simulink model "xz_packaging_automatic"  (R2025b)
settings: Solver=ode15s  StartTime=0.0  StopTime=13.05  MaxStep=0.001  RelTol=1e-6  AbsTol=1e-9
model workspace: external: MATLAB File xz_packaging_automatic_DataFile.m (data not in the file)
values from neighbouring files (symbols this model uses):
  payloadMass_kg = 0.25    [xz_packaging_automatic_DataFile.m]
undefined symbols (not defined in the file or in its folder): smiData, X, Y, Z
libraries: sm_lib x2549, nesl_utility x31
(part 37 of 38)

== system xz_packaging_automatic/Z_AXIS_ELGC_BS_45_200/RigidSubsystem/Z_GUIDE_FIXED_MOUNTS_RIGID/Z_GUIDE_FIXED_MOUNTS_1_RIGID/Z_FGUIDE_RIGHT_FOOT_WASH_1_LOW_RIGID ==
  ReferenceFrame : sm_lib/Frames and Transforms/Reference Frame
  Solid : sm_lib/Body Elements/File Solid  ExtGeomFileName=z_fguide_right_foot_wash_1_low_prt.step  UnitType=FromFile  ExtGeomFileUnits=m  StepReaderType=HEX  ExportConvexHullGeometry=off  InertiaType=Custom  BasedOnType=DensityFromFile  Density=1000  DensityUnits=kg/m^3  Mass=smiData.Solid(88).mass  MassUnits=kg  CenterOfMass=smiData.Solid(88).CoM  CenterOfMassUnits=mm  MomentsOfInertia=smiData.Solid(88).MoI  MomentsOfInertiaUnits=kg*mm^2  ProductsOfInertia=smiData.Solid(88).PoI  ProductsOfInertiaUnits=kg*mm^2  GraphicType=FromGeometry  MarkerShape=Sphere  MarkerSize=10  GraphicVisPropType=SimpleVisualProperties  GraphicDiffuseColor=smiData.Solid(88).color  GraphicOpacity=smiData.Solid(88).opacity  GraphicSpecularColor=[0.5 0.5 0.5 1.0]  GraphicAmbientColor=[0.15 0.15 0.15 1.0]  GraphicEmissiveColor=[0.0 0.0 0.0 1.0]  GraphicShininess=75  DoExposeReferenceFrame=on  SerializedFrames=<Frames/>
  F : PMIOPort  Side=Left
  connections:
  Solid/RConn1 -- ReferenceFrame/RConn1 -- F/RConn1

== system xz_packaging_automatic/Z_AXIS_ELGC_BS_45_200/RigidSubsystem/Z_GUIDE_FIXED_MOUNTS_RIGID/Z_GUIDE_FIXED_MOUNTS_1_RIGID/Z_FGUIDE_RIGHT_FOOT_WASH_1_TOP_RIGID ==
  ReferenceFrame : sm_lib/Frames and Transforms/Reference Frame
  Solid : sm_lib/Body Elements/File Solid  ExtGeomFileName=z_fguide_right_foot_wash_1_top_prt.step  UnitType=FromFile  ExtGeomFileUnits=m  StepReaderType=HEX  ExportConvexHullGeometry=off  InertiaType=Custom  BasedOnType=DensityFromFile  Density=1000  DensityUnits=kg/m^3  Mass=smiData.Solid(87).mass  MassUnits=kg  CenterOfMass=smiData.Solid(87).CoM  CenterOfMassUnits=mm  MomentsOfInertia=smiData.Solid(87).MoI  MomentsOfInertiaUnits=kg*mm^2  ProductsOfInertia=smiData.Solid(87).PoI  ProductsOfInertiaUnits=kg*mm^2  GraphicType=FromGeometry  MarkerShape=Sphere  MarkerSize=10  GraphicVisPropType=SimpleVisualProperties  GraphicDiffuseColor=smiData.Solid(87).color  GraphicOpacity=smiData.Solid(87).opacity  GraphicSpecularColor=[0.5 0.5 0.5 1.0]  GraphicAmbientColor=[0.15 0.15 0.15 1.0]  GraphicEmissiveColor=[0.0 0.0 0.0 1.0]  GraphicShininess=75  DoExposeReferenceFrame=on  SerializedFrames=<Frames/>
  F : PMIOPort  Side=Left
  connections:
  Solid/RConn1 -- ReferenceFrame/RConn1 -- F/RConn1

== system xz_packaging_automatic/Z_AXIS_ELGC_BS_45_200/RigidSubsystem/Z_GUIDE_FIXED_MOUNTS_RIGID/Z_GUIDE_FIXED_MOUNTS_1_RIGID/Z_FGUIDE_RIGHT_FOOT_WASH_2_LOW_RIGID ==
  ReferenceFrame : sm_lib/Frames and Transforms/Reference Frame
  Solid : sm_lib/Body Elements/File Solid  ExtGeomFileName=z_fguide_right_foot_wash_2_low_prt.step  UnitType=FromFile  ExtGeomFileUnits=m  StepReaderType=HEX  ExportConvexHullGeometry=off  InertiaType=Custom  BasedOnType=DensityFromFile  Density=1000  DensityUnits=kg/m^3  Mass=smiData.Solid(96).mass  MassUnits=kg  CenterOfMass=smiData.Solid(96).CoM  CenterOfMassUnits=mm  MomentsOfInertia=smiData.Solid(96).MoI  MomentsOfInertiaUnits=kg*mm^2  ProductsOfInertia=smiData.Solid(96).PoI  ProductsOfInertiaUnits=kg*mm^2  GraphicType=FromGeometry  MarkerShape=Sphere  MarkerSize=10  GraphicVisPropType=SimpleVisualProperties  GraphicDiffuseColor=smiData.Solid(96).color  GraphicOpacity=smiData.Solid(96).opacity  GraphicSpecularColor=[0.5 0.5 0.5 1.0]  GraphicAmbientColor=[0.15 0.15 0.15 1.0]  GraphicEmissiveColor=[0.0 0.0 0.0 1.0]  GraphicShininess=75  DoExposeReferenceFrame=on  SerializedFrames=<Frames/>
  F : PMIOPort  Side=Left
  connections:
  Solid/RConn1 -- ReferenceFrame/RConn1 -- F/RConn1

== system xz_packaging_automatic/Z_AXIS_ELGC_BS_45_200/RigidSubsystem/Z_GUIDE_FIXED_MOUNTS_RIGID/Z_GUIDE_FIXED_MOUNTS_1_RIGID/Z_FGUIDE_RIGHT_FOOT_WASH_2_TOP_RIGID ==
  ReferenceFrame : sm_lib/Frames and Transforms/Reference Frame
  Solid : sm_lib/Body Elements/File Solid  ExtGeomFileName=z_fguide_right_foot_wash_2_top_prt.step  UnitType=FromFile  ExtGeomFileUnits=m  StepReaderType=HEX  ExportConvexHullGeometry=off  InertiaType=Custom  BasedOnType=DensityFromFile  Density=1000  DensityUnits=kg/m^3  Mass=smiData.Solid(95).mass  MassUnits=kg  CenterOfMass=smiData.Solid(95).CoM  CenterOfMassUnits=mm  MomentsOfInertia=smiData.Solid(95).MoI  MomentsOfInertiaUnits=kg*mm^2  ProductsOfInertia=smiData.Solid(95).PoI  ProductsOfInertiaUnits=kg*mm^2  GraphicType=FromGeometry  MarkerShape=Sphere  MarkerSize=10  GraphicVisPropType=SimpleVisualProperties  GraphicDiffuseColor=smiData.Solid(95).color  GraphicOpacity=smiData.Solid(95).opacity  GraphicSpecularColor=[0.5 0.5 0.5 1.0]  GraphicAmbientColor=[0.15 0.15 0.15 1.0]  GraphicEmissiveColor=[0.0 0.0 0.0 1.0]  GraphicShininess=75  DoExposeReferenceFrame=on  SerializedFrames=<Frames/>
  F : PMIOPort  Side=Left
  connections:
  Solid/RConn1 -- ReferenceFrame/RConn1 -- F/RConn1

== system xz_packaging_automatic/Z_AXIS_ELGC_BS_45_200/RigidSubsystem/Z_GUIDE_FIXED_MOUNTS_RIGID/Z_GUIDE_FIXED_MOUNTS_1_RIGID/Z_FGUIDE_RIGHT_WALL_BOLT_1_M3X1_RIGID ==
  ReferenceFrame : sm_lib/Frames and Transforms/Reference Frame
  Solid : sm_lib/Body Elements/File Solid  ExtGeomFileName=z_fguide_right_wall_bolt_1_m3x1_prt.step  UnitType=FromFile  ExtGeomFileUnits=m  StepReaderType=HEX  ExportConvexHullGeometry=off  InertiaType=Custom  BasedOnType=DensityFromFile  Density=1000  DensityUnits=kg/m^3  Mass=smiData.Solid(90).mass  MassUnits=kg  CenterOfMass=smiData.Solid(90).CoM  CenterOfMassUnits=mm  MomentsOfInertia=smiData.Solid(90).MoI  MomentsOfInertiaUnits=kg*mm^2  ProductsOfInertia=smiData.Solid(90).PoI  ProductsOfInertiaUnits=kg*mm^2  GraphicType=FromGeometry  MarkerShape=Sphere  MarkerSize=10  GraphicVisPropType=SimpleVisualProperties  GraphicDiffuseColor=smiData.Solid(90).color  GraphicOpacity=smiData.Solid(90).opacity  GraphicSpecularColor=[0.5 0.5 0.5 1.0]  GraphicAmbientColor=[0.15 0.15 0.15 1.0]  GraphicEmissiveColor=[0.0 0.0 0.0 1.0]  GraphicShininess=75  DoExposeReferenceFrame=on  SerializedFrames=<Frames/>
  F : PMIOPort  Side=Left
  connections:
  Solid/RConn1 -- ReferenceFrame/RConn1 -- F/RConn1

== system xz_packaging_automatic/Z_AXIS_ELGC_BS_45_200/RigidSubsystem/Z_GUIDE_FIXED_MOUNTS_RIGID/Z_GUIDE_FIXED_MOUNTS_1_RIGID/Z_FGUIDE_RIGHT_WALL_BOLT_2_M3X1_RIGID ==
  ReferenceFrame : sm_lib/Frames and Transforms/Reference Frame
  Solid : sm_lib/Body Elements/File Solid  ExtGeomFileName=z_fguide_right_wall_bolt_2_m3x1_prt.step  UnitType=FromFile  ExtGeomFileUnits=m  StepReaderType=HEX  ExportConvexHullGeometry=off  InertiaType=Custom  BasedOnType=DensityFromFile  Density=1000  DensityUnits=kg/m^3  Mass=smiData.Solid(98).mass  MassUnits=kg  CenterOfMass=smiData.Solid(98).CoM  CenterOfMassUnits=mm  MomentsOfInertia=smiData.Solid(98).MoI  MomentsOfInertiaUnits=kg*mm^2  ProductsOfInertia=smiData.Solid(98).PoI  ProductsOfInertiaUnits=kg*mm^2  GraphicType=FromGeometry  MarkerShape=Sphere  MarkerSize=10  GraphicVisPropType=SimpleVisualProperties  GraphicDiffuseColor=smiData.Solid(98).color  GraphicOpacity=smiData.Solid(98).opacity  GraphicSpecularColor=[0.5 0.5 0.5 1.0]  GraphicAmbientColor=[0.15 0.15 0.15 1.0]  GraphicEmissiveColor=[0.0 0.0 0.0 1.0]  GraphicShininess=75  DoExposeReferenceFrame=on  SerializedFrames=<Frames/>
  F : PMIOPort  Side=Left
  connections:
  Solid/RConn1 -- ReferenceFrame/RConn1 -- F/RConn1

== system xz_packaging_automatic/Z_AXIS_ELGC_BS_45_200/RigidSubsystem/Z_GUIDE_FIXED_MOUNTS_RIGID/Z_GUIDE_FIXED_MOUNTS_1_RIGID/Z_FGUIDE_RIGHT_WALL_NUT_1_M3_RIGID ==
  ReferenceFrame : sm_lib/Frames and Transforms/Reference Frame
  Solid : sm_lib/Body Elements/File Solid  ExtGeomFileName=z_fguide_right_wall_nut_1_m3_prt.step  UnitType=FromFile  ExtGeomFileUnits=m  StepReaderType=HEX  ExportConvexHullGeometry=off  InertiaType=Custom  BasedOnType=DensityFromFile  Density=1000  DensityUnits=kg/m^3  Mass=smiData.Solid(93).mass  MassUnits=kg  CenterOfMass=smiData.Solid(93).CoM  CenterOfMassUnits=mm  MomentsOfInertia=smiData.Solid(93).MoI  MomentsOfInertiaUnits=kg*mm^2  ProductsOfInertia=smiData.Solid(93).PoI  ProductsOfInertiaUnits=kg*mm^2  GraphicType=FromGeometry  MarkerShape=Sphere  MarkerSize=10  GraphicVisPropType=SimpleVisualProperties  GraphicDiffuseColor=smiData.Solid(93).color  GraphicOpacity=smiData.Solid(93).opacity  GraphicSpecularColor=[0.5 0.5 0.5 1.0]  GraphicAmbientColor=[0.15 0.15 0.15 1.0]  GraphicEmissiveColor=[0.0 0.0 0.0 1.0]  GraphicShininess=75  DoExposeReferenceFrame=on  SerializedFrames=<Frames/>
  F : PMIOPort  Side=Left
  connections:
  Solid/RConn1 -- ReferenceFrame/RConn1 -- F/RConn1

== system xz_packaging_automatic/Z_AXIS_ELGC_BS_45_200/RigidSubsystem/Z_GUIDE_FIXED_MOUNTS_RIGID/Z_GUIDE_FIXED_MOUNTS_1_RIGID/Z_FGUIDE_RIGHT_WALL_NUT_2_M3_RIGID ==
  ReferenceFrame : sm_lib/Frames and Transforms/Reference Frame
  Solid : sm_lib/Body Elements/File Solid  ExtGeomFileName=z_fguide_right_wall_nut_2_m3_prt.step  UnitType=FromFile  ExtGeomFileUnits=m  StepReaderType=HEX  ExportConvexHullGeometry=off  InertiaType=Custom  BasedOnType=DensityFromFile  Density=1000  DensityUnits=kg/m^3  Mass=smiData.Solid(101).mass  MassUnits=kg  CenterOfMass=smiData.Solid(101).CoM  CenterOfMassUnits=mm  MomentsOfInertia=smiData.Solid(101).MoI  MomentsOfInertiaUnits=kg*mm^2  ProductsOfInertia=smiData.Solid(101).PoI  ProductsOfInertiaUnits=kg*mm^2  GraphicType=FromGeometry  MarkerShape=Sphere  MarkerSize=10  GraphicVisPropType=SimpleVisualProperties  GraphicDiffuseColor=smiData.Solid(101).color  GraphicOpacity=smiData.Solid(101).opacity  GraphicSpecularColor=[0.5 0.5 0.5 1.0]  GraphicAmbientColor=[0.15 0.15 0.15 1.0]  GraphicEmissiveColor=[0.0 0.0 0.0 1.0]  GraphicShininess=75  DoExposeReferenceFrame=on  SerializedFrames=<Frames/>
  F : PMIOPort  Side=Left
  connections:
  Solid/RConn1 -- ReferenceFrame/RConn1 -- F/RConn1

== system xz_packaging_automatic/Z_AXIS_ELGC_BS_45_200/RigidSubsystem/Z_GUIDE_FIXED_MOUNTS_RIGID/Z_GUIDE_FIXED_MOUNTS_1_RIGID/Z_FGUIDE_RIGHT_WALL_WASH_1_INNE_RIGID ==
  ReferenceFrame : sm_lib/Frames and Transforms/Reference Frame
  Solid : sm_lib/Body Elements/File Solid  ExtGeomFileName=z_fguide_right_wall_wash_1_inne_prt.step  UnitType=FromFile  ExtGeomFileUnits=m  StepReaderType=HEX  ExportConvexHullGeometry=off  InertiaType=Custom  BasedOnType=DensityFromFile  Density=1000  DensityUnits=kg/m^3  Mass=smiData.Solid(91).mass  MassUnits=kg  CenterOfMass=smiData.Solid(91).CoM  CenterOfMassUnits=mm  MomentsOfInertia=smiData.Solid(91).MoI  MomentsOfInertiaUnits=kg*mm^2  ProductsOfInertia=smiData.Solid(91).PoI  ProductsOfInertiaUnits=kg*mm^2  GraphicType=FromGeometry  MarkerShape=Sphere  MarkerSize=10  GraphicVisPropType=SimpleVisualProperties  GraphicDiffuseColor=smiData.Solid(91).color  GraphicOpacity=smiData.Solid(91).opacity  GraphicSpecularColor=[0.5 0.5 0.5 1.0]  GraphicAmbientColor=[0.15 0.15 0.15 1.0]  GraphicEmissiveColor=[0.0 0.0 0.0 1.0]  GraphicShininess=75  DoExposeReferenceFrame=on  SerializedFrames=<Frames/>
  F : PMIOPort  Side=Left
  connections:
  Solid/RConn1 -- ReferenceFrame/RConn1 -- F/RConn1

== system xz_packaging_automatic/Z_AXIS_ELGC_BS_45_200/RigidSubsystem/Z_GUIDE_FIXED_MOUNTS_RIGID/Z_GUIDE_FIXED_MOUNTS_1_RIGID/Z_FGUIDE_RIGHT_WALL_WASH_1_OUTE_RIGID ==
  ReferenceFrame : sm_lib/Frames and Transforms/Reference Frame
  Solid : sm_lib/Body Elements/File Solid  ExtGeomFileName=z_fguide_right_wall_wash_1_oute_prt.step  UnitType=FromFile  ExtGeomFileUnits=m  StepReaderType=HEX  ExportConvexHullGeometry=off  InertiaType=Custom  BasedOnType=DensityFromFile  Density=1000  DensityUnits=kg/m^3  Mass=smiData.Solid(92).mass  MassUnits=kg  CenterOfMass=smiData.Solid(92).CoM  CenterOfMassUnits=mm  MomentsOfInertia=smiData.Solid(92).MoI  MomentsOfInertiaUnits=kg*mm^2  ProductsOfInertia=smiData.Solid(92).PoI  ProductsOfInertiaUnits=kg*mm^2  GraphicType=FromGeometry  MarkerShape=Sphere  MarkerSize=10  GraphicVisPropType=SimpleVisualProperties  GraphicDiffuseColor=smiData.Solid(92).color  GraphicOpacity=smiData.Solid(92).opacity  GraphicSpecularColor=[0.5 0.5 0.5 1.0]  GraphicAmbientColor=[0.15 0.15 0.15 1.0]  GraphicEmissiveColor=[0.0 0.0 0.0 1.0]  GraphicShininess=75  DoExposeReferenceFrame=on  SerializedFrames=<Frames/>
  F : PMIOPort  Side=Left
  connections:
  Solid/RConn1 -- ReferenceFrame/RConn1 -- F/RConn1

== system xz_packaging_automatic/Z_AXIS_ELGC_BS_45_200/RigidSubsystem/Z_GUIDE_FIXED_MOUNTS_RIGID/Z_GUIDE_FIXED_MOUNTS_1_RIGID/Z_FGUIDE_RIGHT_WALL_WASH_2_INNE_RIGID ==
  ReferenceFrame : sm_lib/Frames and Transforms/Reference Frame
  Solid : sm_lib/Body Elements/File Solid  ExtGeomFileName=z_fguide_right_wall_wash_2_inne_prt.step  UnitType=FromFile  ExtGeomFileUnits=m  StepReaderType=HEX  ExportConvexHullGeometry=off  InertiaType=Custom  BasedOnType=DensityFromFile  Density=1000  DensityUnits=kg/m^3  Mass=smiData.Solid(99).mass  MassUnits=kg  CenterOfMass=smiData.Solid(99).CoM  CenterOfMassUnits=mm  MomentsOfInertia=smiData.Solid(99).MoI  MomentsOfInertiaUnits=kg*mm^2  ProductsOfInertia=smiData.Solid(99).PoI  ProductsOfInertiaUnits=kg*mm^2  GraphicType=FromGeometry  MarkerShape=Sphere  MarkerSize=10  GraphicVisPropType=SimpleVisualProperties  GraphicDiffuseColor=smiData.Solid(99).color  GraphicOpacity=smiData.Solid(99).opacity  GraphicSpecularColor=[0.5 0.5 0.5 1.0]  GraphicAmbientColor=[0.15 0.15 0.15 1.0]  GraphicEmissiveColor=[0.0 0.0 0.0 1.0]  GraphicShininess=75  DoExposeReferenceFrame=on  SerializedFrames=<Frames/>
  F : PMIOPort  Side=Left
  connections:
  Solid/RConn1 -- ReferenceFrame/RConn1 -- F/RConn1

== system xz_packaging_automatic/Z_AXIS_ELGC_BS_45_200/RigidSubsystem/Z_GUIDE_FIXED_MOUNTS_RIGID/Z_GUIDE_FIXED_MOUNTS_1_RIGID/Z_FGUIDE_RIGHT_WALL_WASH_2_OUTE_RIGID ==
  ReferenceFrame : sm_lib/Frames and Transforms/Reference Frame
  Solid : sm_lib/Body Elements/File Solid  ExtGeomFileName=z_fguide_right_wall_wash_2_oute_prt.step  UnitType=FromFile  ExtGeomFileUnits=m  StepReaderType=HEX  ExportConvexHullGeometry=off  InertiaType=Custom  BasedOnType=DensityFromFile  Density=1000  DensityUnits=kg/m^3  Mass=smiData.Solid(100).mass  MassUnits=kg  CenterOfMass=smiData.Solid(100).CoM  CenterOfMassUnits=mm  MomentsOfInertia=smiData.Solid(100).MoI  MomentsOfInertiaUnits=kg*mm^2  ProductsOfInertia=smiData.Solid(100).PoI  ProductsOfInertiaUnits=kg*mm^2  GraphicType=FromGeometry  MarkerShape=Sphere  MarkerSize=10  GraphicVisPropType=SimpleVisualProperties  GraphicDiffuseColor=smiData.Solid(100).color  GraphicOpacity=smiData.Solid(100).opacity  GraphicSpecularColor=[0.5 0.5 0.5 1.0]  GraphicAmbientColor=[0.15 0.15 0.15 1.0]  GraphicEmissiveColor=[0.0 0.0 0.0 1.0]  GraphicShininess=75  DoExposeReferenceFrame=on  SerializedFrames=<Frames/>
  F : PMIOPort  Side=Left
  connections:
  Solid/RConn1 -- ReferenceFrame/RConn1 -- F/RConn1

== system xz_packaging_automatic/Z_AXIS_ELGC_BS_45_200/RigidSubsystem/Z_GUIDE_FIXED_MOUNTS_RIGID/Z_GUIDE_FIXED_MOUNTS_1_RIGID/Z_FIXED_GUIDE_ANGLE_LEFT_RIGID ==
  ReferenceFrame : sm_lib/Frames and Transforms/Reference Frame
  Solid : sm_lib/Body Elements/File Solid  ExtGeomFileName=z_fixed_guide_angle_left_prt.step  UnitType=FromFile  ExtGeomFileUnits=m  StepReaderType=HEX  ExportConvexHullGeometry=off  InertiaType=Custom  BasedOnType=DensityFromFile  Density=1000  DensityUnits=kg/m^3  Mass=smiData.Solid(85).mass  MassUnits=kg  CenterOfMass=smiData.Solid(85).CoM  CenterOfMassUnits=mm  MomentsOfInertia=smiData.Solid(85).MoI  MomentsOfInertiaUnits=kg*mm^2  ProductsOfInertia=smiData.Solid(85).PoI  ProductsOfInertiaUnits=kg*mm^2  GraphicType=FromGeometry  MarkerShape=Sphere  MarkerSize=10  GraphicVisPropType=SimpleVisualProperties  GraphicDiffuseColor=smiData.Solid(85).color  GraphicOpacity=smiData.Solid(85).opacity  GraphicSpecularColor=[0.5 0.5 0.5 1.0]  GraphicAmbientColor=[0.15 0.15 0.15 1.0]  GraphicEmissiveColor=[0.0 0.0 0.0 1.0]  GraphicShininess=75  DoExposeReferenceFrame=on  SerializedFrames=<Frames/>
  F : PMIOPort  Side=Left
  connections:
  Solid/RConn1 -- ReferenceFrame/RConn1 -- F/RConn1

== system xz_packaging_automatic/Z_AXIS_ELGC_BS_45_200/RigidSubsystem/Z_GUIDE_FIXED_MOUNTS_RIGID/Z_GUIDE_FIXED_MOUNTS_1_RIGID/Z_FIXED_GUIDE_ANGLE_RIGHT_RIGID ==
  ReferenceFrame : sm_lib/Frames and Transforms/Reference Frame
  Solid : sm_lib/Body Elements/File Solid  ExtGeomFileName=z_fixed_guide_angle_right_prt.step  UnitType=FromFile  ExtGeomFileUnits=m  StepReaderType=HEX  ExportConvexHullGeometry=off  InertiaType=Custom  BasedOnType=DensityFromFile  Density=1000  DensityUnits=kg/m^3  Mass=smiData.Solid(103).mass  MassUnits=kg  CenterOfMass=smiData.Solid(103).CoM  CenterOfMassUnits=mm  MomentsOfInertia=smiData.Solid(103).MoI  MomentsOfInertiaUnits=kg*mm^2  ProductsOfInertia=smiData.Solid(103).PoI  ProductsOfInertiaUnits=kg*mm^2  GraphicType=FromGeometry  MarkerShape=Sphere  MarkerSize=10  GraphicVisPropType=SimpleVisualProperties  GraphicDiffuseColor=smiData.Solid(103).color  GraphicOpacity=smiData.Solid(103).opacity  GraphicSpecularColor=[0.5 0.5 0.5 1.0]  GraphicAmbientColor=[0.15 0.15 0.15 1.0]  GraphicEmissiveColor=[0.0 0.0 0.0 1.0]  GraphicShininess=75  DoExposeReferenceFrame=on  SerializedFrames=<Frames/>
  F : PMIOPort  Side=Left
  connections:
  Solid/RConn1 -- ReferenceFrame/RConn1 -- F/RConn1

== system xz_packaging_automatic/Z_AXIS_ELGC_BS_45_200/RigidSubsystem/Z_GUIDE_FIXED_MOUNTS_RIGID/Z_GUIDE_FIXED_MOUNTS_1_RIGID/Z_FIXED_LATERAL_GUIDE_LEFT_RIGID ==
  ReferenceFrame : sm_lib/Frames and Transforms/Reference Frame
  Solid : sm_lib/Body Elements/File Solid  ExtGeomFileName=z_fixed_lateral_guide_left_prt.step  UnitType=FromFile  ExtGeomFileUnits=m  StepReaderType=HEX  ExportConvexHullGeometry=off  InertiaType=Custom  BasedOnType=DensityFromFile  Density=1000  DensityUnits=kg/m^3  Mass=smiData.Solid(84).mass  MassUnits=kg  CenterOfMass=smiData.Solid(84).CoM  CenterOfMassUnits=mm  MomentsOfInertia=smiData.Solid(84).MoI  MomentsOfInertiaUnits=kg*mm^2  ProductsOfInertia=smiData.Solid(84).PoI  ProductsOfInertiaUnits=kg*mm^2  GraphicType=FromGeometry  MarkerShape=Sphere  MarkerSize=10  GraphicVisPropType=SimpleVisualProperties  GraphicDiffuseColor=smiData.Solid(84).color  GraphicOpacity=smiData.Solid(84).opacity  GraphicSpecularColor=[0.5 0.5 0.5 1.0]  GraphicAmbientColor=[0.15 0.15 0.15 1.0]  GraphicEmissiveColor=[0.0 0.0 0.0 1.0]  GraphicShininess=75  DoExposeReferenceFrame=on  SerializedFrames=<Frames/>
  F : PMIOPort  Side=Left
  connections:
  Solid/RConn1 -- ReferenceFrame/RConn1 -- F/RConn1

== system xz_packaging_automatic/Z_AXIS_ELGC_BS_45_200/RigidSubsystem/Z_GUIDE_FIXED_MOUNTS_RIGID/Z_GUIDE_FIXED_MOUNTS_1_RIGID/Z_FIXED_LATERAL_GUIDE_RIGHT_RIGID ==
  ReferenceFrame : sm_lib/Frames and Transforms/Reference Frame
  Solid : sm_lib/Body Elements/File Solid  ExtGeomFileName=z_fixed_lateral_guide_right_prt.step  UnitType=FromFile  ExtGeomFileUnits=m  StepReaderType=HEX  ExportConvexHullGeometry=off  InertiaType=Custom  BasedOnType=DensityFromFile  Density=1000  DensityUnits=kg/m^3  Mass=smiData.Solid(102).mass  MassUnits=kg  CenterOfMass=smiData.Solid(102).CoM  CenterOfMassUnits=mm  MomentsOfInertia=smiData.Solid(102).MoI  MomentsOfInertiaUnits=kg*mm^2  ProductsOfInertia=smiData.Solid(102).PoI  ProductsOfInertiaUnits=kg*mm^2  GraphicType=FromGeometry  MarkerShape=Sphere  MarkerSize=10  GraphicVisPropType=SimpleVisualProperties  GraphicDiffuseColor=smiData.Solid(102).color  GraphicOpacity=smiData.Solid(102).opacity  GraphicSpecularColor=[0.5 0.5 0.5 1.0]  GraphicAmbientColor=[0.15 0.15 0.15 1.0]  GraphicEmissiveColor=[0.0 0.0 0.0 1.0]  GraphicShininess=75  DoExposeReferenceFrame=on  SerializedFrames=<Frames/>
  F : PMIOPort  Side=Left
  connections:
  Solid/RConn1 -- ReferenceFrame/RConn1 -- F/RConn1

== system xz_packaging_automatic/Z_AXIS_ELGC_BS_45_200/RigidSubsystem/Z_SERVICE_FIXED_HARDWARE_RIGID/Z_SERVICE_FIXED_HARDWARE_1_RIGID/Z_BRIDGE_LEFT_BOLT_M3X8_RIGID ==
  ReferenceFrame : sm_lib/Frames and Transforms/Reference Frame
  Solid : sm_lib/Body Elements/File Solid  ExtGeomFileName=z_bridge_left_bolt_m3x8_prt.step  UnitType=FromFile  ExtGeomFileUnits=m  StepReaderType=HEX  ExportConvexHullGeometry=off  InertiaType=Custom  BasedOnType=DensityFromFile  Density=1000  DensityUnits=kg/m^3  Mass=smiData.Solid(64).mass  MassUnits=kg  CenterOfMass=smiData.Solid(64).CoM  CenterOfMassUnits=mm  MomentsOfInertia=smiData.Solid(64).MoI  MomentsOfInertiaUnits=kg*mm^2  ProductsOfInertia=smiData.Solid(64).PoI  ProductsOfInertiaUnits=kg*mm^2  GraphicType=FromGeometry  MarkerShape=Sphere  MarkerSize=10  GraphicVisPropType=SimpleVisualProperties  GraphicDiffuseColor=smiData.Solid(64).color  GraphicOpacity=smiData.Solid(64).opacity  GraphicSpecularColor=[0.5 0.5 0.5 1.0]  GraphicAmbientColor=[0.15 0.15 0.15 1.0]  GraphicEmissiveColor=[0.0 0.0 0.0 1.0]  GraphicShininess=75  DoExposeReferenceFrame=on  SerializedFrames=<Frames/>
  F : PMIOPort  Side=Left
  connections:
  Solid/RConn1 -- ReferenceFrame/RConn1 -- F/RConn1

== system xz_packaging_automatic/Z_AXIS_ELGC_BS_45_200/RigidSubsystem/Z_SERVICE_FIXED_HARDWARE_RIGID/Z_SERVICE_FIXED_HARDWARE_1_RIGID/Z_BRIDGE_LEFT_WASHER_RIGID ==
  ReferenceFrame : sm_lib/Frames and Transforms/Reference Frame
  Solid : sm_lib/Body Elements/File Solid  ExtGeomFileName=z_bridge_left_washer_prt.step  UnitType=FromFile  ExtGeomFileUnits=m  StepReaderType=HEX  ExportConvexHullGeometry=off  InertiaType=Custom  BasedOnType=DensityFromFile  Density=1000  DensityUnits=kg/m^3  Mass=smiData.Solid(65).mass  MassUnits=kg  CenterOfMass=smiData.Solid(65).CoM  CenterOfMassUnits=mm  MomentsOfInertia=smiData.Solid(65).MoI  MomentsOfInertiaUnits=kg*mm^2  ProductsOfInertia=smiData.Solid(65).PoI  ProductsOfInertiaUnits=kg*mm^2  GraphicType=FromGeometry  MarkerShape=Sphere  MarkerSize=10  GraphicVisPropType=SimpleVisualProperties  GraphicDiffuseColor=smiData.Solid(65).color  GraphicOpacity=smiData.Solid(65).opacity  GraphicSpecularColor=[0.5 0.5 0.5 1.0]  GraphicAmbientColor=[0.15 0.15 0.15 1.0]  GraphicEmissiveColor=[0.0 0.0 0.0 1.0]  GraphicShininess=75  DoExposeReferenceFrame=on  SerializedFrames=<Frames/>
  F : PMIOPort  Side=Left
  connections:
  Solid/RConn1 -- ReferenceFrame/RConn1 -- F/RConn1

== system xz_packaging_automatic/Z_AXIS_ELGC_BS_45_200/RigidSubsystem/Z_SERVICE_FIXED_HARDWARE_RIGID/Z_SERVICE_FIXED_HARDWARE_1_RIGID/Z_BRIDGE_RIGHT_BOLT_M3X8_RIGID ==
  ReferenceFrame : sm_lib/Frames and Transforms/Reference Frame
  Solid : sm_lib/Body Elements/File Solid  ExtGeomFileName=z_bridge_right_bolt_m3x8_prt.step  UnitType=FromFile  ExtGeomFileUnits=m  StepReaderType=HEX  ExportConvexHullGeometry=off  InertiaType=Custom  BasedOnType=DensityFromFile  Density=1000  DensityUnits=kg/m^3  Mass=smiData.Solid(66).mass  MassUnits=kg  CenterOfMass=smiData.Solid(66).CoM  CenterOfMassUnits=mm  MomentsOfInertia=smiData.Solid(66).MoI  MomentsOfInertiaUnits=kg*mm^2  ProductsOfInertia=smiData.Solid(66).PoI  ProductsOfInertiaUnits=kg*mm^2  GraphicType=FromGeometry  MarkerShape=Sphere  MarkerSize=10  GraphicVisPropType=SimpleVisualProperties  GraphicDiffuseColor=smiData.Solid(66).color  GraphicOpacity=smiData.Solid(66).opacity  GraphicSpecularColor=[0.5 0.5 0.5 1.0]  GraphicAmbientColor=[0.15 0.15 0.15 1.0]  GraphicEmissiveColor=[0.0 0.0 0.0 1.0]  GraphicShininess=75  DoExposeReferenceFrame=on  SerializedFrames=<Frames/>
  F : PMIOPort  Side=Left
  connections:
  Solid/RConn1 -- ReferenceFrame/RConn1 -- F/RConn1

== system xz_packaging_automatic/Z_AXIS_ELGC_BS_45_200/RigidSubsystem/Z_SERVICE_FIXED_HARDWARE_RIGID/Z_SERVICE_FIXED_HARDWARE_1_RIGID/Z_BRIDGE_RIGHT_WASHER_RIGID ==
  ReferenceFrame : sm_lib/Frames and Transforms/Reference Frame
  Solid : sm_lib/Body Elements/File Solid  ExtGeomFileName=z_bridge_right_washer_prt.step  UnitType=FromFile  ExtGeomFileUnits=m  StepReaderType=HEX  ExportConvexHullGeometry=off  InertiaType=Custom  BasedOnType=DensityFromFile  Density=1000  DensityUnits=kg/m^3  Mass=smiData.Solid(67).mass  MassUnits=kg  CenterOfMass=smiData.Solid(67).CoM  CenterOfMassUnits=mm  MomentsOfInertia=smiData.Solid(67).MoI  MomentsOfInertiaUnits=kg*mm^2  ProductsOfInertia=smiData.Solid(67).PoI  ProductsOfInertiaUnits=kg*mm^2  GraphicType=FromGeometry  MarkerShape=Sphere  MarkerSize=10  GraphicVisPropType=SimpleVisualProperties  GraphicDiffuseColor=smiData.Solid(67).color  GraphicOpacity=smiData.Solid(67).opacity  GraphicSpecularColor=[0.5 0.5 0.5 1.0]  GraphicAmbientColor=[0.15 0.15 0.15 1.0]  GraphicEmissiveColor=[0.0 0.0 0.0 1.0]  GraphicShininess=75  DoExposeReferenceFrame=on  SerializedFrames=<Frames/>
  F : PMIOPort  Side=Left
  connections:
  Solid/RConn1 -- ReferenceFrame/RConn1 -- F/RConn1

== system xz_packaging_automatic/Z_AXIS_ELGC_BS_45_200/RigidSubsystem/Z_SERVICE_FIXED_HARDWARE_RIGID/Z_SERVICE_FIXED_HARDWARE_1_RIGID/Z_COLLAR_FRONT_BOLT_M3X60_RIGID ==
  ReferenceFrame : sm_lib/Frames and Transforms/Reference Frame
  Solid : sm_lib/Body Elements/File Solid  ExtGeomFileName=z_collar_front_bolt_m3x60_prt.step  UnitType=FromFile  ExtGeomFileUnits=m  StepReaderType=HEX  ExportConvexHullGeometry=off  InertiaType=Custom  BasedOnType=DensityFromFile  Density=1000  DensityUnits=kg/m^3  Mass=smiData.Solid(60).mass  MassUnits=kg  CenterOfMass=smiData.Solid(60).CoM  CenterOfMassUnits=mm  MomentsOfInertia=smiData.Solid(60).MoI  MomentsOfInertiaUnits=kg*mm^2  ProductsOfInertia=smiData.Solid(60).PoI  ProductsOfInertiaUnits=kg*mm^2  GraphicType=FromGeometry  MarkerShape=Sphere  MarkerSize=10  GraphicVisPropType=SimpleVisualProperties  GraphicDiffuseColor=smiData.Solid(60).color  GraphicOpacity=smiData.Solid(60).opacity  GraphicSpecularColor=[0.5 0.5 0.5 1.0]  GraphicAmbientColor=[0.15 0.15 0.15 1.0]  GraphicEmissiveColor=[0.0 0.0 0.0 1.0]  GraphicShininess=75  DoExposeReferenceFrame=on  SerializedFrames=<Frames/>
  F : PMIOPort  Side=Left
  connections:
  Solid/RConn1 -- ReferenceFrame/RConn1 -- F/RConn1

== system xz_packaging_automatic/Z_AXIS_ELGC_BS_45_200/RigidSubsystem/Z_SERVICE_FIXED_HARDWARE_RIGID/Z_SERVICE_FIXED_HARDWARE_1_RIGID/Z_COLLAR_FRONT_NUT_M3_RIGID ==
  ReferenceFrame : sm_lib/Frames and Transforms/Reference Frame
  Solid : sm_lib/Body Elements/File Solid  ExtGeomFileName=z_collar_front_nut_m3_prt.step  UnitType=FromFile  ExtGeomFileUnits=m  StepReaderType=HEX  ExportConvexHullGeometry=off  InertiaType=Custom  BasedOnType=DensityFromFile  Density=1000  DensityUnits=kg/m^3  Mass=smiData.Solid(63).mass  MassUnits=kg  CenterOfMass=smiData.Solid(63).CoM  CenterOfMassUnits=mm  MomentsOfInertia=smiData.Solid(63).MoI  MomentsOfInertiaUnits=kg*mm^2  ProductsOfInertia=smiData.Solid(63).PoI  ProductsOfInertiaUnits=kg*mm^2  GraphicType=FromGeometry  MarkerShape=Sphere  MarkerSize=10  GraphicVisPropType=SimpleVisualProperties  GraphicDiffuseColor=smiData.Solid(63).color  GraphicOpacity=smiData.Solid(63).opacity  GraphicSpecularColor=[0.5 0.5 0.5 1.0]  GraphicAmbientColor=[0.15 0.15 0.15 1.0]  GraphicEmissiveColor=[0.0 0.0 0.0 1.0]  GraphicShininess=75  DoExposeReferenceFrame=on  SerializedFrames=<Frames/>
  F : PMIOPort  Side=Left
  connections:
  Solid/RConn1 -- ReferenceFrame/RConn1 -- F/RConn1

== system xz_packaging_automatic/Z_AXIS_ELGC_BS_45_200/RigidSubsystem/Z_SERVICE_FIXED_HARDWARE_RIGID/Z_SERVICE_FIXED_HARDWARE_1_RIGID/Z_COLLAR_FRONT_WASHER_LEFT_RIGID ==
  ReferenceFrame : sm_lib/Frames and Transforms/Reference Frame
  Solid : sm_lib/Body Elements/File Solid  ExtGeomFileName=z_collar_front_washer_left_prt.step  UnitType=FromFile  ExtGeomFileUnits=m  StepReaderType=HEX  ExportConvexHullGeometry=off  InertiaType=Custom  BasedOnType=DensityFromFile  Density=1000  DensityUnits=kg/m^3  Mass=smiData.Solid(61).mass  MassUnits=kg  CenterOfMass=smiData.Solid(61).CoM  CenterOfMassUnits=mm  MomentsOfInertia=smiData.Solid(61).MoI  MomentsOfInertiaUnits=kg*mm^2  ProductsOfInertia=smiData.Solid(61).PoI  ProductsOfInertiaUnits=kg*mm^2  GraphicType=FromGeometry  MarkerShape=Sphere  MarkerSize=10  GraphicVisPropType=SimpleVisualProperties  GraphicDiffuseColor=smiData.Solid(61).color  GraphicOpacity=smiData.Solid(61).opacity  GraphicSpecularColor=[0.5 0.5 0.5 1.0]  GraphicAmbientColor=[0.15 0.15 0.15 1.0]  GraphicEmissiveColor=[0.0 0.0 0.0 1.0]  GraphicShininess=75  DoExposeReferenceFrame=on  SerializedFrames=<Frames/>
  F : PMIOPort  Side=Left
  connections:
  Solid/RConn1 -- ReferenceFrame/RConn1 -- F/RConn1

== system xz_packaging_automatic/Z_AXIS_ELGC_BS_45_200/RigidSubsystem/Z_SERVICE_FIXED_HARDWARE_RIGID/Z_SERVICE_FIXED_HARDWARE_1_RIGID/Z_COLLAR_FRONT_WASHER_RIGHT_RIGID ==
  ReferenceFrame : sm_lib/Frames and Transforms/Reference Frame
  Solid : sm_lib/Body Elements/File Solid  ExtGeomFileName=z_collar_front_washer_right_prt.step  UnitType=FromFile  ExtGeomFileUnits=m  StepReaderType=HEX  ExportConvexHullGeometry=off  InertiaType=Custom  BasedOnType=DensityFromFile  Density=1000  DensityUnits=kg/m^3  Mass=smiData.Solid(62).mass  MassUnits=kg  CenterOfMass=smiData.Solid(62).CoM  CenterOfMassUnits=mm  MomentsOfInertia=smiData.Solid(62).MoI  MomentsOfInertiaUnits=kg*mm^2  ProductsOfInertia=smiData.Solid(62).PoI  ProductsOfInertiaUnits=kg*mm^2  GraphicType=FromGeometry  MarkerShape=Sphere  MarkerSize=10  GraphicVisPropType=SimpleVisualProperties  GraphicDiffuseColor=smiData.Solid(62).color  GraphicOpacity=smiData.Solid(62).opacity  GraphicSpecularColor=[0.5 0.5 0.5 1.0]  GraphicAmbientColor=[0.15 0.15 0.15 1.0]  GraphicEmissiveColor=[0.0 0.0 0.0 1.0]  GraphicShininess=75  DoExposeReferenceFrame=on  SerializedFrames=<Frames/>
  F : PMIOPort  Side=Left
  connections:
  Solid/RConn1 -- ReferenceFrame/RConn1 -- F/RConn1

== system xz_packaging_automatic/Z_AXIS_ELGC_BS_45_200/RigidSubsystem/Z_SERVICE_FIXED_HARDWARE_RIGID/Z_SERVICE_FIXED_HARDWARE_1_RIGID/Z_COLLAR_REAR_BOLT_M3X60_RIGID ==
  ReferenceFrame : sm_lib/Frames and Transforms/Reference Frame
  Solid : sm_lib/Body Elements/File Solid  ExtGeomFileName=z_collar_rear_bolt_m3x60_prt.step  UnitType=FromFile  ExtGeomFileUnits=m  StepReaderType=HEX  ExportConvexHullGeometry=off  InertiaType=Custom  BasedOnType=DensityFromFile  Density=1000  DensityUnits=kg/m^3  Mass=smiData.Solid(56).mass  MassUnits=kg  CenterOfMass=smiData.Solid(56).CoM  CenterOfMassUnits=mm  MomentsOfInertia=smiData.Solid(56).MoI  MomentsOfInertiaUnits=kg*mm^2  ProductsOfInertia=smiData.Solid(56).PoI  ProductsOfInertiaUnits=kg*mm^2  GraphicType=FromGeometry  MarkerShape=Sphere  MarkerSize=10  GraphicVisPropType=SimpleVisualProperties  GraphicDiffuseColor=smiData.Solid(56).color  GraphicOpacity=smiData.Solid(56).opacity  GraphicSpecularColor=[0.5 0.5 0.5 1.0]  GraphicAmbientColor=[0.15 0.15 0.15 1.0]  GraphicEmissiveColor=[0.0 0.0 0.0 1.0]  GraphicShininess=75  DoExposeReferenceFrame=on  SerializedFrames=<Frames/>
  F : PMIOPort  Side=Left
  connections:
  Solid/RConn1 -- ReferenceFrame/RConn1 -- F/RConn1

== system xz_packaging_automatic/Z_AXIS_ELGC_BS_45_200/RigidSubsystem/Z_SERVICE_FIXED_HARDWARE_RIGID/Z_SERVICE_FIXED_HARDWARE_1_RIGID/Z_COLLAR_REAR_NUT_M3_RIGID ==
  ReferenceFrame : sm_lib/Frames and Transforms/Reference Frame
  Solid : sm_lib/Body Elements/File Solid  ExtGeomFileName=z_collar_rear_nut_m3_prt.step  UnitType=FromFile  ExtGeomFileUnits=m  StepReaderType=HEX  ExportConvexHullGeometry=off  InertiaType=Custom  BasedOnType=DensityFromFile  Density=1000  DensityUnits=kg/m^3  Mass=smiData.Solid(59).mass  MassUnits=kg  CenterOfMass=smiData.Solid(59).CoM  CenterOfMassUnits=mm  MomentsOfInertia=smiData.Solid(59).MoI  MomentsOfInertiaUnits=kg*mm^2  ProductsOfInertia=smiData.Solid(59).PoI  ProductsOfInertiaUnits=kg*mm^2  GraphicType=FromGeometry  MarkerShape=Sphere  MarkerSize=10  GraphicVisPropType=SimpleVisualProperties  GraphicDiffuseColor=smiData.Solid(59).color  GraphicOpacity=smiData.Solid(59).opacity  GraphicSpecularColor=[0.5 0.5 0.5 1.0]  GraphicAmbientColor=[0.15 0.15 0.15 1.0]  GraphicEmissiveColor=[0.0 0.0 0.0 1.0]  GraphicShininess=75  DoExposeReferenceFrame=on  SerializedFrames=<Frames/>
  F : PMIOPort  Side=Left
  connections:
  Solid/RConn1 -- ReferenceFrame/RConn1 -- F/RConn1

== system xz_packaging_automatic/Z_AXIS_ELGC_BS_45_200/RigidSubsystem/Z_SERVICE_FIXED_HARDWARE_RIGID/Z_SERVICE_FIXED_HARDWARE_1_RIGID/Z_COLLAR_REAR_WASHER_LEFT_RIGID ==
  ReferenceFrame : sm_lib/Frames and Transforms/Reference Frame
  Solid : sm_lib/Body Elements/File Solid  ExtGeomFileName=z_collar_rear_washer_left_prt.step  UnitType=FromFile  ExtGeomFileUnits=m  StepReaderType=HEX  ExportConvexHullGeometry=off  InertiaType=Custom  BasedOnType=DensityFromFile  Density=1000  DensityUnits=kg/m^3  Mass=smiData.Solid(57).mass  MassUnits=kg  CenterOfMass=smiData.Solid(57).CoM  CenterOfMassUnits=mm  MomentsOfInertia=smiData.Solid(57).MoI  MomentsOfInertiaUnits=kg*mm^2  ProductsOfInertia=smiData.Solid(57).PoI  ProductsOfInertiaUnits=kg*mm^2  GraphicType=FromGeometry  MarkerShape=Sphere  MarkerSize=10  GraphicVisPropType=SimpleVisualProperties  GraphicDiffuseColor=smiData.Solid(57).color  GraphicOpacity=smiData.Solid(57).opacity  GraphicSpecularColor=[0.5 0.5 0.5 1.0]  GraphicAmbientColor=[0.15 0.15 0.15 1.0]  GraphicEmissiveColor=[0.0 0.0 0.0 1.0]  GraphicShininess=75  DoExposeReferenceFrame=on  SerializedFrames=<Frames/>
  F : PMIOPort  Side=Left
  connections:
  Solid/RConn1 -- ReferenceFrame/RConn1 -- F/RConn1

== system xz_packaging_automatic/Z_AXIS_ELGC_BS_45_200/RigidSubsystem/Z_SERVICE_FIXED_HARDWARE_RIGID/Z_SERVICE_FIXED_HARDWARE_1_RIGID/Z_COLLAR_REAR_WASHER_RIGHT_RIGID ==
  ReferenceFrame : sm_lib/Frames and Transforms/Reference Frame
  Solid : sm_lib/Body Elements/File Solid  ExtGeomFileName=z_collar_rear_washer_right_prt.step  UnitType=FromFile  ExtGeomFileUnits=m  StepReaderType=HEX  ExportConvexHullGeometry=off  InertiaType=Custom  BasedOnType=DensityFromFile  Density=1000  DensityUnits=kg/m^3  Mass=smiData.Solid(58).mass  MassUnits=kg  CenterOfMass=smiData.Solid(58).CoM  CenterOfMassUnits=mm  MomentsOfInertia=smiData.Solid(58).MoI  MomentsOfInertiaUnits=kg*mm^2  ProductsOfInertia=smiData.Solid(58).PoI  ProductsOfInertiaUnits=kg*mm^2  GraphicType=FromGeometry  MarkerShape=Sphere  MarkerSize=10  GraphicVisPropType=SimpleVisualProperties  GraphicDiffuseColor=smiData.Solid(58).color  GraphicOpacity=smiData.Solid(58).opacity  GraphicSpecularColor=[0.5 0.5 0.5 1.0]  GraphicAmbientColor=[0.15 0.15 0.15 1.0]  GraphicEmissiveColor=[0.0 0.0 0.0 1.0]  GraphicShininess=75  DoExposeReferenceFrame=on  SerializedFrames=<Frames/>
  F : PMIOPort  Side=Left
  connections:
  Solid/RConn1 -- ReferenceFrame/RConn1 -- F/RConn1

== system xz_packaging_automatic/Z_AXIS_ELGC_BS_45_200/RigidSubsystem/Z_SERVICE_FIXED_HARDWARE_RIGID/Z_SERVICE_FIXED_HARDWARE_1_RIGID/Z_SERVICE_ANCHOR_BRIDGE_RIGID ==
  ReferenceFrame : sm_lib/Frames and Transforms/Reference Frame
  Solid : sm_lib/Body Elements/File Solid  ExtGeomFileName=z_service_anchor_bridge_prt.step  UnitType=FromFile  ExtGeomFileUnits=m  StepReaderType=HEX  ExportConvexHullGeometry=off  InertiaType=Custom  BasedOnType=DensityFromFile  Density=1000  DensityUnits=kg/m^3  Mass=smiData.Solid(55).mass  MassUnits=kg  CenterOfMass=smiData.Solid(55).CoM  CenterOfMassUnits=mm  MomentsOfInertia=smiData.Solid(55).MoI  MomentsOfInertiaUnits=kg*mm^2  ProductsOfInertia=smiData.Solid(55).PoI  ProductsOfInertiaUnits=kg*mm^2  GraphicType=FromGeometry  MarkerShape=Sphere  MarkerSize=10  GraphicVisPropType=SimpleVisualProperties  GraphicDiffuseColor=smiData.Solid(55).color  GraphicOpacity=smiData.Solid(55).opacity  GraphicSpecularColor=[0.5 0.5 0.5 1.0]  GraphicAmbientColor=[0.15 0.15 0.15 1.0]  GraphicEmissiveColor=[0.0 0.0 0.0 1.0]  GraphicShininess=75  DoExposeReferenceFrame=on  SerializedFrames=<Frames/>
  F : PMIOPort  Side=Left
  connections:
  Solid/RConn1 -- ReferenceFrame/RConn1 -- F/RConn1

== system xz_packaging_automatic/Z_AXIS_ELGC_BS_45_200/RigidSubsystem/Z_SERVICE_FIXED_HARDWARE_RIGID/Z_SERVICE_FIXED_HARDWARE_1_RIGID/Z_SERVICE_COLLAR_LEFT_RIGID ==
  ReferenceFrame : sm_lib/Frames and Transforms/Reference Frame
  Solid : sm_lib/Body Elements/File Solid  ExtGeomFileName=z_service_collar_left_prt.step  UnitType=FromFile  ExtGeomFileUnits=m  StepReaderType=HEX  ExportConvexHullGeometry=off  InertiaType=Custom  BasedOnType=DensityFromFile  Density=1000  DensityUnits=kg/m^3  Mass=smiData.Solid(53).mass  MassUnits=kg  CenterOfMass=smiData.Solid(53).CoM  CenterOfMassUnits=mm  MomentsOfInertia=smiData.Solid(53).MoI  MomentsOfInertiaUnits=kg*mm^2  ProductsOfInertia=smiData.Solid(53).PoI  ProductsOfInertiaUnits=kg*mm^2  GraphicType=FromGeometry  MarkerShape=Sphere  MarkerSize=10  GraphicVisPropType=SimpleVisualProperties  GraphicDiffuseColor=smiData.Solid(53).color  GraphicOpacity=smiData.Solid(53).opacity  GraphicSpecularColor=[0.5 0.5 0.5 1.0]  GraphicAmbientColor=[0.15 0.15 0.15 1.0]  GraphicEmissiveColor=[0.0 0.0 0.0 1.0]  GraphicShininess=75  DoExposeReferenceFrame=on  SerializedFrames=<Frames/>
  F : PMIOPort  Side=Left
  connections:
  Solid/RConn1 -- ReferenceFrame/RConn1 -- F/RConn1

== system xz_packaging_automatic/Z_AXIS_ELGC_BS_45_200/RigidSubsystem/Z_SERVICE_FIXED_HARDWARE_RIGID/Z_SERVICE_FIXED_HARDWARE_1_RIGID/Z_SERVICE_COLLAR_RIGHT_RIGID ==
  ReferenceFrame : sm_lib/Frames and Transforms/Reference Frame
  Solid : sm_lib/Body Elements/File Solid  ExtGeomFileName=z_service_collar_right_prt.step  UnitType=FromFile  ExtGeomFileUnits=m  StepReaderType=HEX  ExportConvexHullGeometry=off  InertiaType=Custom  BasedOnType=DensityFromFile  Density=1000  DensityUnits=kg/m^3  Mass=smiData.Solid(54).mass  MassUnits=kg  CenterOfMass=smiData.Solid(54).CoM  CenterOfMassUnits=mm  MomentsOfInertia=smiData.Solid(54).MoI  MomentsOfInertiaUnits=kg*mm^2  ProductsOfInertia=smiData.Solid(54).PoI  ProductsOfInertiaUnits=kg*mm^2  GraphicType=FromGeometry  MarkerShape=Sphere  MarkerSize=10  GraphicVisPropType=SimpleVisualProperties  GraphicDiffuseColor=smiData.Solid(54).color  GraphicOpacity=smiData.Solid(54).opacity  GraphicSpecularColor=[0.5 0.5 0.5 1.0]  GraphicAmbientColor=[0.15 0.15 0.15 1.0]  GraphicEmissiveColor=[0.0 0.0 0.0 1.0]  GraphicShininess=75  DoExposeReferenceFrame=on  SerializedFrames=<Frames/>
  F : PMIOPort  Side=Left
  connections:
  Solid/RConn1 -- ReferenceFrame/RConn1 -- F/RConn1

== matlab function xz_packaging_automatic/Select axis forces ==
  data: enabled input; force output; x input; z input; q input; v input; owner input; contact input; external input; service input; raw output; limited output; refLog output; payload input
function [force,raw,limited,refLog] = selectForce(enabled,x,z,q,v,owner,contact,external,service,payload)
persistent integral
if isempty(integral)
    integral = zeros(2,1);
end
p.empty_mass_kg = [7.1948956018947463;0.89277415808894123];
p.gravity_m_s2 = 9.8066499999999994;
p.kp_N_m = [15342.440856384694;2355.0289849896903];
p.kd_N_s_m = [562.83410750324276;86.393726351523952];
p.ki_N_m_s = [137224.31573412396;21063.613281895363];
p.force_limit_N = [35;35];
p.sample_time_s = 0.001;
p.antiwindup_s_inv = 25;
refLog = [x z]';
if enabled>0.5
    carriedMass = payload*double(owner==2);
    vNow = v+p.sample_time_s*refLog(:,3);
    qNow = q+0.5*p.sample_time_s*(v+vNow);
    [limited,integral,raw] = axis_control_step(refLog,qNow,vNow,carriedMass,sum(contact),integral,p);
else
    raw = external;
    limited = external;
    integral(:) = 0;
end
force = limited+min(10,max(-10,service));
end

function [command, integralNext, raw] = axis_control_step(ref,q,v,carriedMass,contactN,integral,p)
% Order X, Z; ref columns are position, velocity and acceleration in SI.
% contactN is the upward normal force from both cups, positive in magnitude.
mass = p.empty_mass_kg(:)+carriedMass;
feedforward = mass.*ref(:,3);
feedforward(2) = feedforward(2)-mass(2)*p.gravity_m_s2+contactN;
error = ref(:,1)-q;
raw = feedforward + p.kp_N_m(:).*error + p.kd_N_s_m(:).*(ref(:,2)-v) + integral;
limit = p.force_limit_N(:);
command = min(limit,max(-limit,raw));
integralNext = integral+p.sample_time_s*(p.ki_N_m_s(:).*error+p.antiwindup_s_inv*(command-raw));
end

== matlab function xz_packaging_automatic/Belt travel to drums and phase ==
  data: s input; infeed output; outfeed output; phase output
function [infeed,outfeed,phase] = belt_mapping(s)
% Travel is positive in each conveyor's process direction.
infeed = reshape(s(1:3),3,1)/0.02725;
outfeed = -reshape(s(4:6),3,1)/0.02725;
phase = mod([s(1);s(4)],1.2592167996206438);
end

== matlab function xz_packaging_automatic/Demo process inputs ==
  data: t input; process output; stage input; entered input
function process = demo_supply(t,stage,entered)
% External supplier/receiver mock. Start, then acknowledge each new exchange.
age = t-entered;
process = [double(t>=0.02);0;0; ...
    double(stage==20 && age>=0.15);double(stage==20 && age>=0.25); ...
    double(stage==24 && age>=0.20);0;1;1;1;0;1];
end

== matlab function xz_packaging_automatic/VACUUM_GRIP_COMPONENTS/right normal contact ==
  data: qZ input; force output; vZ input; height input; compression input; speed input; enabled input
function force = contact(qZ,vZ,height,compression,speed,enabled)
penetration = qZ - 0.17400000000000002 + height - compression;
depth = enabled*max(0,penetration);
engagement = min(1,depth/0.00002);
force = max(0,100000*depth + 35*engagement*(vZ-speed));
end

== matlab function xz_packaging_automatic/VACUUM_GRIP_COMPONENTS/left normal contact ==
  data: qZ input; force output; vZ input; height input; compression input; speed input; enabled input
function force = contact(qZ,vZ,height,compression,speed,enabled)
penetration = qZ - 0.17400000000000002 + height - compression;
depth = enabled*max(0,penetration);
engagement = min(1,depth/0.00002);
force = max(0,100000*depth + 35*engagement*(vZ-speed));
end

== matlab function xz_packaging_automatic/Vacuum interlocks ==
  data: t input; stage output; dL input; dR input; fL input; fR input; process input; start output; pressure output; owner output; vacuum output; seat output; q input; v input; travel input; cycle output; holdPose output; stations output; axisReference input
function [stage,start,pressure,owner,vacuum,seat,cycle,holdPose,stations] = automatic_process(t,dL,dR,fL,fR,process,q,v,travel,axisReference)
% process = [start stop reset supplyCarton supplyCarrier unload leak inReady outReady axesReady ventBlocked settlePermit].
% Travel uses positive process direction on each belt.
% 1 ms bench interlock. Owner: 1 = infeed, 2 = tool, 3 = outfeed.
persistent phase entered dp readySince count fault last seen fed carried hold holdVac base parked followingSince
if isempty(phase)
    phase = 0;
    entered = 0;
    dp = zeros(2,1);
    readySince = -1;
    count = 0;
    fault = 0;
    last = zeros(5,1);
    seen = false(2,1);
    fed = false;
    carried = 1;
    hold = [0.05;0.024;0;0];
    holdVac = false;
    base = zeros(2,1);
    parked = false;
    followingSince = -1;
end
elapsed = t-entered;
process = process(:);
rising = process([1 3 4 5 6])>0.5 & last<=0.5;
last = process([1 3 4 5 6]);
registered = fed && abs(travel(2)-base(2)-0.015)<=0.0005;
productAtPick = fed && abs(travel(1)-base(1)-0.16)<=0.0005;
leakRight = process(7);
atPick = abs(q(1)-0.05)<=0.00005;
atDrop = abs(q(1)-0.45)<=0.00005;
seatLeft = dL>=0.0005 && dL<=0.002 && fL>2;
seatRight = dR>=0.0005 && dR<=0.002 && fR>2;
seat = seatLeft && seatRight && fL+fR<=10;
energized = phase>=2 && phase<=7 || (phase==90 && holdVac);
holdingSeal = phase>=3 && phase<=7 || (phase==90 && holdVac);
target = zeros(2,1);
tau = 0.06;
if energized
    target = 5000 + 55000*double([seatLeft || holdingSeal; seatRight || holdingSeal]);
    if leakRight > 0.5
        target(2) = min(target(2),25000);
    end
    tau = 0.10;
end
if t > 0 && ~(phase==8 && process(11)>0.5) && ~(phase==90 && fault==4)
    dp = target + (dp-target)*exp(-0.001/tau);
end
next = phase;
stopped = all(abs(v)<=0.005);
raised = abs(q(2)-0.024)<=0.00005;
atHome = atPick && raised && stopped;
ready = false;
switch phase
    case 1
        ready = elapsed>=2.15 && atPick && abs(q(2)-0.1755)<=0.00005 && stopped;
    case 3
        ready = elapsed>=0.30 && atPick && abs(q(2)-0.174)<=0.00005 && stopped;
    case 4
        ready = elapsed>=1 && atPick && abs(q(2)-0.024)<=0.00005 && stopped;
    case 5
        ready = elapsed>=1.30 && atDrop && registered && abs(q(2)-0.024)<=0.00005 && stopped;
    case 6
        ready = elapsed>=1.80 && atDrop && registered && abs(q(2)-0.174)<=0.00005 && stopped;
    case 7
        ready = elapsed>=0.40 && atDrop && registered && seat && abs(q(2)-0.1755)<=0.00005 && stopped;
    case 9
        ready = elapsed>=1.30 && atDrop && abs(q(2)-0.024)<=0.00005 && stopped;
    case 21
        ready = elapsed>=1 && abs(travel(1)-base(1)-0.16)<=0.0005 && ...
            abs(travel(2)-base(2)-0.015)<=0.0005 && atHome;
    case 22
        ready = elapsed>=1 && abs(travel(2)-base(2)-0.175)<=0.0005 && atDrop && raised && stopped;
    case 23
        ready = elapsed>=1.30 && atHome;
    case 12
        ready = elapsed>=1.30 && atPick && abs(q(2)-0.024)<=0.00005 && stopped;
end
ready = ready && (phase==21 || phase==22 || process(12)>0.5);
if ~ready
    readySince = -1;
elseif readySince<0
    readySince = t;
end
settled = readySince>=0 && t-readySince>=0.05;
switch phase
    case 0
        if rising(1) && atHome && process(10)>0.5
            next = 20;
        end
    case 20
        seen = seen | rising(3:4);
        if all(seen) && atHome && process(10)>0.5
            next = 21;
            fed = true;
            parked = false;
        end
    case 21
        if settled
            next = 1;
        elseif elapsed>=1.60
            fault = 2;
        end
    case 1
        if settled
            next = 2;
        end
    case 2
        if seat && atPick && productAtPick && elapsed>=0.10 && all(dp>=58000)
            next = 3;
        elseif elapsed>=0.60
            next = 11;
            fault = 1;
        end
    case 3
        if settled
            next = 4;
        end
    case 4
        if settled
            next = 5;
        end
    case 5
        if settled
            next = 6;
        end
    case 6
        if settled
            next = 7;
        end
    case 7
        if settled
            next = 8;
        elseif elapsed>=1.20
            fault = 3;
        end
    case 8
        if ~registered || ~atDrop || ~seat
            fault = 3;
        elseif elapsed>=0.08 && all(dp<=5000) && process(2)<=0.5 && process(10)>0.5
            next = 9;
            count = count+1;
        elseif elapsed>=0.50
            fault = 4;
        end
    case 9
        if settled
            next = 22;
        end
    case 22
        if settled
            next = 24;
        elseif elapsed>=1.60
            fault = 2;
        end
    case 24
        if rising(5)
            next = 23;
        elseif elapsed>=2.0
            fault = 5;
        end
    case 23
        if settled
            next = 20;
            base = base+[0.16;0.175];
            fed = false;
            seen(:) = false;
            parked = true;
        end
    case 13
        if rising(2) && atHome && ~any(process(4:5)>0.5)
            next = 0;
            fault = 0;
            fed = false;
            base = travel;
            seen(:) = false;
        end
    case 90
        if rising(2) && atHome && carried==1 && ~holdVac && ~any(process(4:5)>0.5)
            next = 0;
            fault = 0;
            fed = false;
            base = travel;
            seen(:) = false;
        end
    case 11
        if all(dp<=5000)
            next = 12;
        end
    case 12
        if settled
            next = 13;
        end
end
axisTimeout = (phase==1 && elapsed>2.65) || (phase==3 && elapsed>0.80) || ...
    (phase==4 && elapsed>1.50) || (phase==5 && elapsed>1.80) || ...
    (phase==6 && elapsed>2.30) || (phase==7 && elapsed>1.20) || ...
    ((phase==9 || phase==12 || phase==23) && elapsed>1.80);
axisMoving = any(phase==[1 3 4 5 6 7 9 12 23]);
if axisMoving && any(abs(q-axisReference(:,1))>0.002)
    if followingSince<0
        followingSince = t;
    end
else
    followingSince = -1;
end
if phase~=90 && phase~=13
    if process(2)>0.5
        fault = 6;
    elseif process(10)<=0.5 && phase~=0 && phase~=20 || axisTimeout
        fault = 3;
    elseif (phase==21 || phase==22) && abs(q(2)-0.024)>0.0005
        fault = 3;
    elseif phase>=4 && phase<=6 && any(dp<58000)
        fault = 7;
    elseif followingSince>=0 && t-followingSince>=0.020
        fault = 8;
    end
    if fault~=0 && (fault~=1 || axisTimeout)
        next = 90;
        hold = [q;travel];
        carried = ownership(phase,parked);
        holdVac = phase>=2 && phase<=7;
    end
end
if next~=phase
    phase = next;
    entered = t;
    readySince = -1;
end
stage = phase;
start = entered;
pressure = dp;
owner = ownership(stage,parked);
if stage==90
    owner = carried;
end
vacuum = double(stage>=2 && stage<=7 || (stage==90 && holdVac));
cycle = [count;fault;double(stage==20 && count>0);base;double(fed); ...
    double(process(8)>0.5);double(process(9)>0.5);double(parked)];
holdPose = hold;
stations = [double(productAtPick);double(registered);travel(2)-base(2)-0.015;leakRight];
end

function owner = ownership(stage,parked)
owner = 1;
if stage>=4 && stage<=6
    owner = 2;
elseif (stage>=7 && stage<=9) || any(stage==[22 23 24]) || (stage==20 && parked)
    owner = 3;
end
end
